simulink model "im_inv_model"  (R2026a)
settings: Solver=ode23tb  StopTime=param.sim.simlength  FixedStep=param.sim.tc  MaxStep=param.glb_time.tc  EnableMultiTasking=on
values from neighbouring files (symbols this model uses):
  param = struct()    [init_model.m]
undefined symbols (not defined in the file or in its folder): magnitude
libraries: fl_lib x53, nesl_utility x25, simulink x2, lithium_ion_battery x1, induction_machine x1, threephase_inductor_lib x1, dclink_with_center_tap x1, cstblocks_lti x1
(part 2 of 3)

== system im_inv_model/inverter//ctrl/im_ctrl/abc2dq  ==
  a : Inport
  b : Inport  Port=2
  c : Inport  Port=3
  wt : Inport  Port=4
  abc2alphabeta : Subsystem
  alphabeta2dq : Subsystem
  d : Outport  VectorParamsAs1DForOutWhenUnconnected=off
  q : Outport  Port=2  VectorParamsAs1DForOutWhenUnconnected=off
  wires:
  alphabeta2dq/2(q) -> q/1
  alphabeta2dq/1(d) -> d/1
  a/1 -> abc2alphabeta/1(a)
  c/1 -> abc2alphabeta/3(c)
  b/1 -> abc2alphabeta/2(b)
  wt/1 -> alphabeta2dq/3(wt)
  abc2alphabeta/2("beta ") -> alphabeta2dq/2(beta)
  abc2alphabeta/1("alpha ") -> alphabeta2dq/1(alpha)

== system im_inv_model/inverter//ctrl/im_ctrl/acquisition ==
  Demux1 : Demux  Outputs=3
  Gain4 : Gain  Gain=1/param.im.machine.ibez
  Gain5 : Gain  Gain=1/param.im.machine.ibez
  Gain6 : Gain  Gain=1/param.im.machine.ibez
  Quantizer1 : Quantizer  QuantizationInterval=param.meas.adc12_quantization
  Quantizer2 : Quantizer  QuantizationInterval=param.meas.adc12_quantization
  Quantizer3 : Quantizer  QuantizationInterval=param.meas.adc12_quantization
  Zero-Order Hold : ZeroOrderHold  SampleTime=param.glb_time.ts_inv
  Zero-Order Hold1 : ZeroOrderHold  SampleTime=param.glb_time.ts_inv
  Zero-Order Hold2 : ZeroOrderHold  SampleTime=param.glb_time.ts_inv
  iu : Outport  VectorParamsAs1DForOutWhenUnconnected=off
  iv : Outport  Port=2  VectorParamsAs1DForOutWhenUnconnected=off
  iw : Outport  Port=3  VectorParamsAs1DForOutWhenUnconnected=off
  wires:
  Demux1/1 -> Gain4/1
  Demux1/2 -> Gain5/1
  Demux1/3 -> Gain6/1
  [is_uvw_mod1] -> Demux1/1
  Quantizer3/1 -> Zero-Order Hold/1
  Quantizer1/1 -> Zero-Order Hold1/1
  Quantizer2/1 -> Zero-Order Hold2/1
  Gain4/1 -> Quantizer3/1
  Gain5/1 -> Quantizer1/1
  Gain6/1 -> Quantizer2/1
  Zero-Order Hold/1 -> iu/1
  Zero-Order Hold1/1 -> iv/1
  Zero-Order Hold2/1 -> iw/1

== system im_inv_model/inverter//ctrl/im_ctrl/dq2alphabeta ==
  x : Inport
  y : Inport  Port=2
  theta_s : Inport  Port=3
  dq-alphabeta : Subsystem
  dq-alphabeta1 : Subsystem
  uctrl_alpha : Outport  VectorParamsAs1DForOutWhenUnconnected=off
  uctrl_beta : Outport  Port=2  VectorParamsAs1DForOutWhenUnconnected=off
  tag scope: uctrl_alpha_mod1=global, uctrl_beta_mod1=global, ud_inv_mod1=global, uq_inv_mod1=global
  wires:
  x/1 -> dq-alphabeta/2(d), dq-alphabeta1/2(d)
  y/1 -> dq-alphabeta/3(q), dq-alphabeta1/3(q)
  theta_s/1 -> dq-alphabeta/1(wt)
  dq-alphabeta/1(alpha) -> [uctrl_alpha_mod1], uctrl_alpha/1
  dq-alphabeta/2(beta) -> [uctrl_beta_mod1], uctrl_beta/1
  [theta_slip_mod1] -> dq-alphabeta1/1(wt)
  dq-alphabeta1/1(alpha) -> [ud_inv_mod1]
  dq-alphabeta1/2(beta) -> [uq_inv_mod1]

== system im_inv_model/inverter//ctrl/im_ctrl/im_control ==
  Constant : Constant  Value=param.im.machine.alpha_norm
  Speed control : Subsystem
  Variant Source : VariantSource  VariantControls={param.im.mode.use_vector_control == 1, param.im.mode.use_uf_control == 1}
      settings: AllowZeroVariantControls=on
  Variant Source1 : VariantSource  VariantControls={param.im.mode.use_vector_control == 1, param.im.mode.use_uf_control == 1}
      settings: AllowZeroVariantControls=on
  Variant Source2 : VariantSource  VariantControls={param.im.mode.use_vector_control == 1, param.im.mode.use_uf_control == 1}
      settings: AllowZeroVariantControls=on
  current control : Subsystem
  data_analysis : Subsystem
  flux_estimator : Subsystem
  magnetization current reference : Subsystem
  speed reference : Subsystem
  u/f control : Subsystem
  usx : Outport  VectorParamsAs1DForOutWhenUnconnected=off
  usy : Outport  Port=2  VectorParamsAs1DForOutWhenUnconnected=off
  theta_s : Outport  Port=3  VectorParamsAs1DForOutWhenUnconnected=off
  tag scope: theta_s_mod1=global, torque_ref_pu_mod1=global
  wires:
  magnetization current reference/1(Ix_ref) -> current control/1(isx_ref)
  magnetization current reference/2(Iy_ref) -> current control/2(isy_ref)
  Speed control/1(torque ref) -> [torque_ref_pu_mod1]
  [omega_m_pu_mod1] -> Speed control/1(Rotor speed)
  speed reference/1(omega_m_pu_ref) -> Speed control/2(Speed ref)
  Constant/1 -> flux_estimator/1(alpha_est)
  current control/1(usx_ctrl) -> Variant Source/1
  current control/2(usy_ctrl) -> Variant Source1/1
  Variant Source/1 -> usx/1
  Variant Source1/1 -> usy/1
  u/f control/1(usx_ctrl) -> Variant Source/2
  u/f control/2(usy_ctrl) -> Variant Source1/2
  flux_estimator/1(theta_s) -> [theta_s_mod1]
  [theta_s_mod1] -> Variant Source2/1
  u/f control/3(uf_electrical_phase) -> Variant Source2/2
  Variant Source2/1 -> theta_s/1

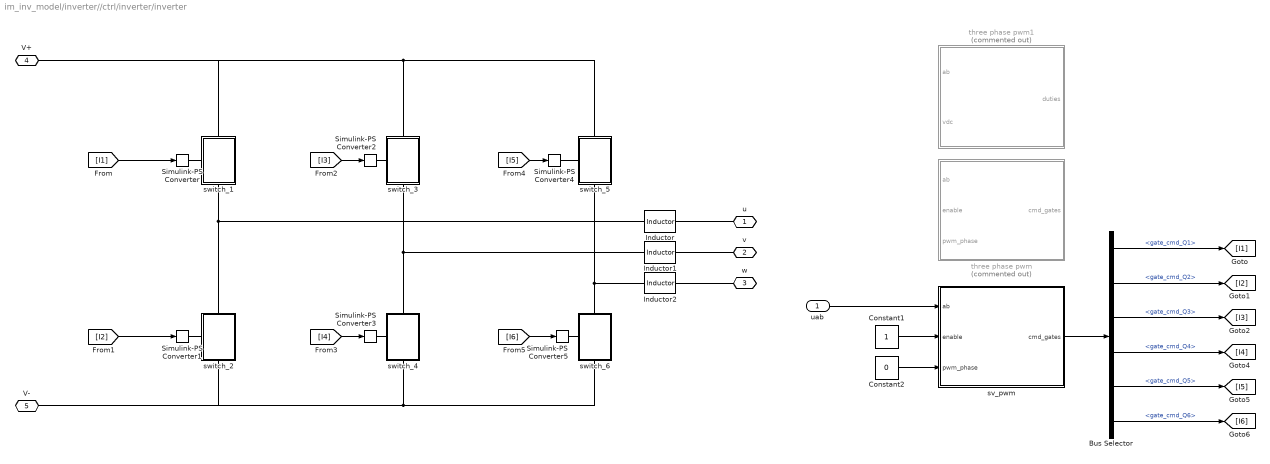
== system im_inv_model/inverter//ctrl/inverter/inverter ==
  uab : Inport
  Bus Selector : BusSelector  OutputSignals=gate_cmd_Q1,gate_cmd_Q2,gate_cmd_Q3,gate_cmd_Q4,gate_cmd_Q5,gate_cmd_Q6
  Constant1 : Constant
  Constant2 : Constant  Value=0
  Inductor : fl_lib/Electrical/Electrical Elements/Inductor  l=1e-6 H  r=0 Ohm  g=1e-9 1/Ohm  i_specify=off  i_priority=None  i=0 A  i_nominal_specify=off  i_nominal_value=1  i_nominal_unit=A  v_specify=off  v_priority=None  v=0 V  v_nominal_specify=off  v_nominal_value=1  v_nominal_unit=V  i_L_specify=off  i_L_priority=High  i_L=0 A  i_L_nominal_specify=off  i_L_nominal_value=1  i_L_nominal_unit=A
  Inductor1 : fl_lib/Electrical/Electrical Elements/Inductor  l=1e-6 H  r=0 Ohm  g=1e-9 1/Ohm  i_specify=off  i_priority=None  i=0 A  i_nominal_specify=off  i_nominal_value=1  i_nominal_unit=A  v_specify=off  v_priority=None  v=0 V  v_nominal_specify=off  v_nominal_value=1  v_nominal_unit=V  i_L_specify=off  i_L_priority=High  i_L=0 A  i_L_nominal_specify=off  i_L_nominal_value=1  i_L_nominal_unit=A
  Inductor2 : fl_lib/Electrical/Electrical Elements/Inductor  l=1e-6 H  r=0 Ohm  g=1e-9 1/Ohm  i_specify=off  i_priority=None  i=0 A  i_nominal_specify=off  i_nominal_value=1  i_nominal_unit=A  v_specify=off  v_priority=None  v=0 V  v_nominal_specify=off  v_nominal_value=1  v_nominal_unit=V  i_L_specify=off  i_L_priority=High  i_L=0 A  i_L_nominal_specify=off  i_L_nominal_value=1  i_L_nominal_unit=A
  Simulink-PS Converter{,1..5} (6 alike) : nesl_utility/Simulink-PS Converter  PhysicalDomain=network_engine_domain  SubClassName=ps_input  LeftPortType=input  RightPortType=output  PseudoPeriodic=off  Frequencies=[]  NoiseDistribution=none  NoiseParameters=[]  Unit=1  AffineConversion=on  FilteringAndDerivatives=provide  SimscapeFilterOrder=1  InputFilterTimeConstant=0.001  UdotUserProvided=0
  sv_pwm : Subsystem
  switch_1 : Subsystem
      settings: PortSchema="{\"entries\":[{\"content\":{\"sides\":[{\"content\":{\"connectorIds\":[\"LConn1\"]},\"type\":\"ConnectorPlacement.EquallySpacedRectSide\",\"uuid\":\"9277da8d-d460-43e6-8478-dd662f15d226\"},{\"content\":{\"connectorIds\":[],\"side\":\"RIGHT\"},\"type\":\"ConnectorPlacement.EquallySpacedRectSide\",\"uuid\":\"a7ece396-f1d9-4f4f-a05b-db1fc65d6e1d\"},{\"content\":{\"connectorIds\":[\"LConn2\"],\"side\":\"TOP\"},\"type\":\"ConnectorPlacement.EquallySpacedRectSide\",\"uuid\":\"fdd70777-e9cf-4317-afb6-cae87f75d5b0\"},{\"content\":{\"connectorIds\":[\"RConn1\"],\"side\":\"BOTTOM\"},\"type\":\"ConnectorPlacement.EquallySpacedRectSide\",\"uuid\":\"2353ed68-b1a1-4775-9ca9-31e268d5443b\"}]},\"type\":\"ConnectorPlacement.EquallySpacedConnector\",\"uuid\":\"d5479f4c-4e65-4791-adcb-73df11f88590\"}],\"packageUris\":[\"http://schema.mathworks.com/mf0/Connector/R2020b\"],\"version\":\"1.0\"}"
  switch_2 : Subsystem
      settings: PortSchema="{\"entries\":[{\"content\":{\"sides\":[{\"content\":{\"connectorIds\":[\"LConn1\"]},\"type\":\"ConnectorPlacement.EquallySpacedRectSide\",\"uuid\":\"9277da8d-d460-43e6-8478-dd662f15d226\"},{\"content\":{\"connectorIds\":[],\"side\":\"RIGHT\"},\"type\":\"ConnectorPlacement.EquallySpacedRectSide\",\"uuid\":\"a7ece396-f1d9-4f4f-a05b-db1fc65d6e1d\"},{\"content\":{\"connectorIds\":[\"LConn2\"],\"side\":\"TOP\"},\"type\":\"ConnectorPlacement.EquallySpacedRectSide\",\"uuid\":\"fdd70777-e9cf-4317-afb6-cae87f75d5b0\"},{\"content\":{\"connectorIds\":[\"RConn1\"],\"side\":\"BOTTOM\"},\"type\":\"ConnectorPlacement.EquallySpacedRectSide\",\"uuid\":\"2353ed68-b1a1-4775-9ca9-31e268d5443b\"}]},\"type\":\"ConnectorPlacement.EquallySpacedConnector\",\"uuid\":\"d5479f4c-4e65-4791-adcb-73df11f88590\"}],\"packageUris\":[\"http://schema.mathworks.com/mf0/Connector/R2020b\"],\"version\":\"1.0\"}"
  switch_3 : Subsystem
      settings: PortSchema="{\"entries\":[{\"content\":{\"sides\":[{\"content\":{\"connectorIds\":[\"LConn1\"]},\"type\":\"ConnectorPlacement.EquallySpacedRectSide\",\"uuid\":\"9277da8d-d460-43e6-8478-dd662f15d226\"},{\"content\":{\"connectorIds\":[],\"side\":\"RIGHT\"},\"type\":\"ConnectorPlacement.EquallySpacedRectSide\",\"uuid\":\"a7ece396-f1d9-4f4f-a05b-db1fc65d6e1d\"},{\"content\":{\"connectorIds\":[\"LConn2\"],\"side\":\"TOP\"},\"type\":\"ConnectorPlacement.EquallySpacedRectSide\",\"uuid\":\"fdd70777-e9cf-4317-afb6-cae87f75d5b0\"},{\"content\":{\"connectorIds\":[\"RConn1\"],\"side\":\"BOTTOM\"},\"type\":\"ConnectorPlacement.EquallySpacedRectSide\",\"uuid\":\"2353ed68-b1a1-4775-9ca9-31e268d5443b\"}]},\"type\":\"ConnectorPlacement.EquallySpacedConnector\",\"uuid\":\"d5479f4c-4e65-4791-adcb-73df11f88590\"}],\"packageUris\":[\"http://schema.mathworks.com/mf0/Connector/R2020b\"],\"version\":\"1.0\"}"
  switch_4 : Subsystem
      settings: PortSchema="{\"entries\":[{\"content\":{\"sides\":[{\"content\":{\"connectorIds\":[\"LConn1\"]},\"type\":\"ConnectorPlacement.EquallySpacedRectSide\",\"uuid\":\"9277da8d-d460-43e6-8478-dd662f15d226\"},{\"content\":{\"connectorIds\":[],\"side\":\"RIGHT\"},\"type\":\"ConnectorPlacement.EquallySpacedRectSide\",\"uuid\":\"a7ece396-f1d9-4f4f-a05b-db1fc65d6e1d\"},{\"content\":{\"connectorIds\":[\"LConn2\"],\"side\":\"TOP\"},\"type\":\"ConnectorPlacement.EquallySpacedRectSide\",\"uuid\":\"fdd70777-e9cf-4317-afb6-cae87f75d5b0\"},{\"content\":{\"connectorIds\":[\"RConn1\"],\"side\":\"BOTTOM\"},\"type\":\"ConnectorPlacement.EquallySpacedRectSide\",\"uuid\":\"2353ed68-b1a1-4775-9ca9-31e268d5443b\"}]},\"type\":\"ConnectorPlacement.EquallySpacedConnector\",\"uuid\":\"d5479f4c-4e65-4791-adcb-73df11f88590\"}],\"packageUris\":[\"http://schema.mathworks.com/mf0/Connector/R2020b\"],\"version\":\"1.0\"}"
  switch_5 : Subsystem
      settings: PortSchema="{\"entries\":[{\"content\":{\"sides\":[{\"content\":{\"connectorIds\":[\"LConn1\"]},\"type\":\"ConnectorPlacement.EquallySpacedRectSide\",\"uuid\":\"9277da8d-d460-43e6-8478-dd662f15d226\"},{\"content\":{\"connectorIds\":[],\"side\":\"RIGHT\"},\"type\":\"ConnectorPlacement.EquallySpacedRectSide\",\"uuid\":\"a7ece396-f1d9-4f4f-a05b-db1fc65d6e1d\"},{\"content\":{\"connectorIds\":[\"LConn2\"],\"side\":\"TOP\"},\"type\":\"ConnectorPlacement.EquallySpacedRectSide\",\"uuid\":\"fdd70777-e9cf-4317-afb6-cae87f75d5b0\"},{\"content\":{\"connectorIds\":[\"RConn1\"],\"side\":\"BOTTOM\"},\"type\":\"ConnectorPlacement.EquallySpacedRectSide\",\"uuid\":\"2353ed68-b1a1-4775-9ca9-31e268d5443b\"}]},\"type\":\"ConnectorPlacement.EquallySpacedConnector\",\"uuid\":\"d5479f4c-4e65-4791-adcb-73df11f88590\"}],\"packageUris\":[\"http://schema.mathworks.com/mf0/Connector/R2020b\"],\"version\":\"1.0\"}"
  switch_6 : Subsystem
      settings: PortSchema="{\"entries\":[{\"content\":{\"sides\":[{\"content\":{\"connectorIds\":[\"LConn1\"]},\"type\":\"ConnectorPlacement.EquallySpacedRectSide\",\"uuid\":\"9277da8d-d460-43e6-8478-dd662f15d226\"},{\"content\":{\"connectorIds\":[],\"side\":\"RIGHT\"},\"type\":\"ConnectorPlacement.EquallySpacedRectSide\",\"uuid\":\"a7ece396-f1d9-4f4f-a05b-db1fc65d6e1d\"},{\"content\":{\"connectorIds\":[\"LConn2\"],\"side\":\"TOP\"},\"type\":\"ConnectorPlacement.EquallySpacedRectSide\",\"uuid\":\"fdd70777-e9cf-4317-afb6-cae87f75d5b0\"},{\"content\":{\"connectorIds\":[\"RConn1\"],\"side\":\"BOTTOM\"},\"type\":\"ConnectorPlacement.EquallySpacedRectSide\",\"uuid\":\"2353ed68-b1a1-4775-9ca9-31e268d5443b\"}]},\"type\":\"ConnectorPlacement.EquallySpacedConnector\",\"uuid\":\"d5479f4c-4e65-4791-adcb-73df11f88590\"}],\"packageUris\":[\"http://schema.mathworks.com/mf0/Connector/R2020b\"],\"version\":\"1.0\"}"
  three phase pwm : Subsystem  Commented=on
  three phase pwm1 : Subsystem  Commented=on
  u : PMIOPort  Side=Left
  v : PMIOPort  Port=2  Side=Left
  w : PMIOPort  Port=3  Side=Left
  V+ : PMIOPort  Port=4  Side=Right
  V- : PMIOPort  Port=5  Side=Right
  wires:
  Bus Selector/6 -> [I6]  "<gate_cmd_Q6>"
  Bus Selector/5 -> [I5]  "<gate_cmd_Q5>"
  Bus Selector/4 -> [I4]  "<gate_cmd_Q4>"
  Bus Selector/3 -> [I3]  "<gate_cmd_Q3>"
  Bus Selector/2 -> [I2]  "<gate_cmd_Q2>"
  Bus Selector/1 -> [I1]  "<gate_cmd_Q1>"
  sv_pwm/1(cmd_gates) -> Bus Selector/1
  [I6] -> Simulink-PS Converter5/1
  [I5] -> Simulink-PS Converter4/1
  [I4] -> Simulink-PS Converter3/1
  [I3] -> Simulink-PS Converter2/1
  uab/1 -> sv_pwm/1(ab)
  Constant2/1 -> sv_pwm/3(pwm_phase)
  Constant1/1 -> sv_pwm/2(enable)
  [I1] -> Simulink-PS Converter/1
  [I2] -> Simulink-PS Converter1/1
  connections:
  V+/RConn1 -- switch_1/LConn2 -- switch_5/LConn2 -- switch_3/LConn2
  Inductor2/LConn1 -- switch_6/LConn2 -- switch_5/RConn1
  Inductor1/LConn1 -- switch_4/LConn2 -- switch_3/RConn1
  u/RConn1 -- Inductor/RConn1
  switch_6/LConn1 -- Simulink-PS Converter5/RConn1
  switch_5/LConn1 -- Simulink-PS Converter4/RConn1
  switch_4/LConn1 -- Simulink-PS Converter3/RConn1
  switch_3/LConn1 -- Simulink-PS Converter2/RConn1
  switch_2/LConn1 -- Simulink-PS Converter1/RConn1
  Simulink-PS Converter/RConn1 -- switch_1/LConn1
  switch_2/RConn1 -- V-/RConn1 -- switch_6/RConn1 -- switch_4/RConn1
  Inductor/LConn1 -- switch_2/LConn2 -- switch_1/RConn1
  v/RConn1 -- Inductor1/RConn1
  w/RConn1 -- Inductor2/RConn1

== system im_inv_model/inverter//ctrl/im_ctrl/abc2dq/abc2alphabeta ==
  a : Inport
  b : Inport  Port=2
  c : Inport  Port=3
  Gain1 : Gain  Gain=-1/2
  Gain11 : Gain  Gain=-1/2
  Gain2 : Gain  Gain=0
  Gain3 : Gain  Gain=sqrt(3)/2
  Gain4 : Gain  Gain=-sqrt(3)/2
  Gain8 : Gain  Gain=2/3
  Gain9 : Gain  Gain=2/3
  Sum : Sum  Inputs=+++
  Sum1 : Sum  Inputs=+++
  "alpha " : Outport  VectorParamsAs1DForOutWhenUnconnected=off
  "beta " : Outport  Port=2  VectorParamsAs1DForOutWhenUnconnected=off
  wires:
  Sum1/1 -> Gain9/1
  Sum/1 -> Gain8/1
  b/1 -> Gain11/1, Gain3/1
  c/1 -> Gain1/1, Gain4/1
  a/1 -> Sum/1, Gain2/1
  Gain4/1 -> Sum1/3
  Gain3/1 -> Sum1/2
  Gain2/1 -> Sum1/1
  Gain8/1 -> "alpha "/1
  Gain9/1 -> "beta "/1
  Gain1/1 -> Sum/3
  Gain11/1 -> Sum/2

== system im_inv_model/inverter//ctrl/im_ctrl/abc2dq/alphabeta2dq ==
  alpha : Inport
  beta : Inport  Port=2
  wt : Inport  Port=3
  Gain : Gain
  Gain1 : Gain
  Product{,1..3} (4 alike) : Product  RndMeth=Zero
  Sum : Sum
  Sum1 : Sum  Inputs=-+
  Trigonometric Function : Trigonometry  Operator=cos
  Trigonometric Function1 : Trigonometry
  d : Outport  VectorParamsAs1DForOutWhenUnconnected=off
  q : Outport  Port=2  VectorParamsAs1DForOutWhenUnconnected=off
  wires:
  [cos] -> Product/1
  alpha/1 -> Product/2, Product2/2
  Product/1 -> Sum/1
  Product1/1 -> Sum/2
  [sin] -> Product1/1
  beta/1 -> Product1/2, Product3/2
  Sum/1 -> Gain/1
  [sin] -> Product2/1
  Product2/1 -> Sum1/1
  Product3/1 -> Sum1/2
  [cos] -> Product3/1
  Sum1/1 -> Gain1/1
  Gain/1 -> d/1
  Gain1/1 -> q/1
  Trigonometric Function1/1 -> [sin]
  Trigonometric Function/1 -> [cos]
  wt/1 -> Trigonometric Function/1, Trigonometric Function1/1

== system im_inv_model/inverter//ctrl/im_ctrl/abc2dq /abc2alphabeta ==
  a : Inport
  b : Inport  Port=2
  c : Inport  Port=3
  Gain1 : Gain  Gain=-1/2
  Gain11 : Gain  Gain=-1/2
  Gain2 : Gain  Gain=0
  Gain3 : Gain  Gain=sqrt(3)/2
  Gain4 : Gain  Gain=-sqrt(3)/2
  Gain8 : Gain  Gain=2/3
  Gain9 : Gain  Gain=2/3
  Sum : Sum  Inputs=+++
  Sum1 : Sum  Inputs=+++
  "alpha " : Outport  VectorParamsAs1DForOutWhenUnconnected=off
  "beta " : Outport  Port=2  VectorParamsAs1DForOutWhenUnconnected=off
  wires:
  Gain11/1 -> Sum/2
  Gain1/1 -> Sum/3
  Gain9/1 -> "beta "/1
  Gain8/1 -> "alpha "/1
  Gain2/1 -> Sum1/1
  Gain3/1 -> Sum1/2
  Gain4/1 -> Sum1/3
  a/1 -> Gain2/1, Sum/1
  c/1 -> Gain4/1, Gain1/1
  b/1 -> Gain3/1, Gain11/1
  Sum/1 -> Gain8/1
  Sum1/1 -> Gain9/1

== system im_inv_model/inverter//ctrl/im_ctrl/abc2dq /alphabeta2dq ==
  alpha : Inport
  beta : Inport  Port=2
  wt : Inport  Port=3
  Gain : Gain
  Gain1 : Gain
  Product{,1..3} (4 alike) : Product  RndMeth=Zero
  Sum : Sum
  Sum1 : Sum  Inputs=-+
  Trigonometric Function : Trigonometry  Operator=cos
  Trigonometric Function1 : Trigonometry
  d : Outport  VectorParamsAs1DForOutWhenUnconnected=off
  q : Outport  Port=2  VectorParamsAs1DForOutWhenUnconnected=off
  wires:
  wt/1 -> Trigonometric Function1/1, Trigonometric Function/1
  Trigonometric Function/1 -> [cos]
  Trigonometric Function1/1 -> [sin]
  Gain1/1 -> q/1
  Gain/1 -> d/1
  Sum1/1 -> Gain1/1
  [cos] -> Product3/1
  Product3/1 -> Sum1/2
  Product2/1 -> Sum1/1
  [sin] -> Product2/1
  Sum/1 -> Gain/1
  beta/1 -> Product3/2, Product1/2
  [sin] -> Product1/1
  Product1/1 -> Sum/2
  Product/1 -> Sum/1
  alpha/1 -> Product2/2, Product/2
  [cos] -> Product/1

== system im_inv_model/inverter//ctrl/im_ctrl/dq2alphabeta/dq-alphabeta ==
  wt : Inport
  d : Inport  Port=2
  q : Inport  Port=3
  Product{,1..3} (4 alike) : Product  RndMeth=Zero
  Sum : Sum  Inputs=+-
  Sum1 : Sum
  Trigonometric Function : Trigonometry  Operator=cos
  Trigonometric Function1 : Trigonometry
  alpha : Outport  VectorParamsAs1DForOutWhenUnconnected=off
  beta : Outport  Port=2  VectorParamsAs1DForOutWhenUnconnected=off
  wires:
  Sum1/1 -> beta/1
  [cos] -> Product3/1
  Product3/1 -> Sum1/2
  Product2/1 -> Sum1/1
  [sin] -> Product2/1
  Sum/1 -> alpha/1
  q/1 -> Product1/2, Product3/2
  [sin] -> Product1/1
  Product1/1 -> Sum/2
  Product/1 -> Sum/1
  d/1 -> Product/2, Product2/2
  [cos] -> Product/1
  Trigonometric Function1/1 -> [sin]
  Trigonometric Function/1 -> [cos]
  wt/1 -> Trigonometric Function/1, Trigonometric Function1/1

== system im_inv_model/inverter//ctrl/im_ctrl/dq2alphabeta/dq-alphabeta1 ==
  wt : Inport
  d : Inport  Port=2
  q : Inport  Port=3
  Product{,1..3} (4 alike) : Product  RndMeth=Zero
  Sum : Sum  Inputs=+-
  Sum1 : Sum
  Trigonometric Function : Trigonometry  Operator=cos
  Trigonometric Function1 : Trigonometry
  alpha : Outport  VectorParamsAs1DForOutWhenUnconnected=off
  beta : Outport  Port=2  VectorParamsAs1DForOutWhenUnconnected=off
  wires:
  wt/1 -> Trigonometric Function1/1, Trigonometric Function/1
  Trigonometric Function/1 -> [cos]
  Trigonometric Function1/1 -> [sin]
  [cos] -> Product/1
  d/1 -> Product/2, Product2/2
  Product/1 -> Sum/1
  Product1/1 -> Sum/2
  [sin] -> Product1/1
  q/1 -> Product1/2, Product3/2
  Sum/1 -> alpha/1
  [sin] -> Product2/1
  Product2/1 -> Sum1/1
  Product3/1 -> Sum1/2
  [cos] -> Product3/1
  Sum1/1 -> beta/1

== system im_inv_model/inverter//ctrl/im_ctrl/im_control/Speed control ==
  Rotor speed : Inport
  Speed ref : Inport  Port=2
  1/Ti : Gain  Gain=param.im.ctrl.kp_w  SaturateOnIntegerOverflow=on  OutDataTypeStr=Inherit: Same as input  ParamDataTypeStr=Inherit: Same as input
  Saturation : Saturate  UpperLimit=param.im.ctrl.iq_lim  LowerLimit=-param.im.ctrl.iq_lim
  Sum1 : Sum  Inputs=+++  SaturateOnIntegerOverflow=on
  Sum2 : Sum  Inputs=-+  SaturateOnIntegerOverflow=on
  Sum3 : Sum  Inputs=-+  SaturateOnIntegerOverflow=on
  Unit Delay4 : UnitDelay  SampleTime=param.glb_time.ts_inv
  kp : Gain  Gain=param.im.ctrl.ki_w*param.glb_time.ts_inv  SaturateOnIntegerOverflow=on  OutDataTypeStr=Inherit: Same as input  ParamDataTypeStr=Inherit: Same as input
  torque ref : Outport  VectorParamsAs1DForOutWhenUnconnected=off
  wires:
  1/Ti/1 -> Sum3/1, Sum1/1
  kp/1 -> Sum1/2
  Sum2/1 -> 1/Ti/1, kp/1
  Sum1/1 -> Saturation/1
  Sum3/1 -> Unit Delay4/1
  Unit Delay4/1 -> Sum1/3
  Speed ref/1 -> Sum2/2
  Rotor speed/1 -> Sum2/1
  Saturation/1 -> torque ref/1, Sum3/2

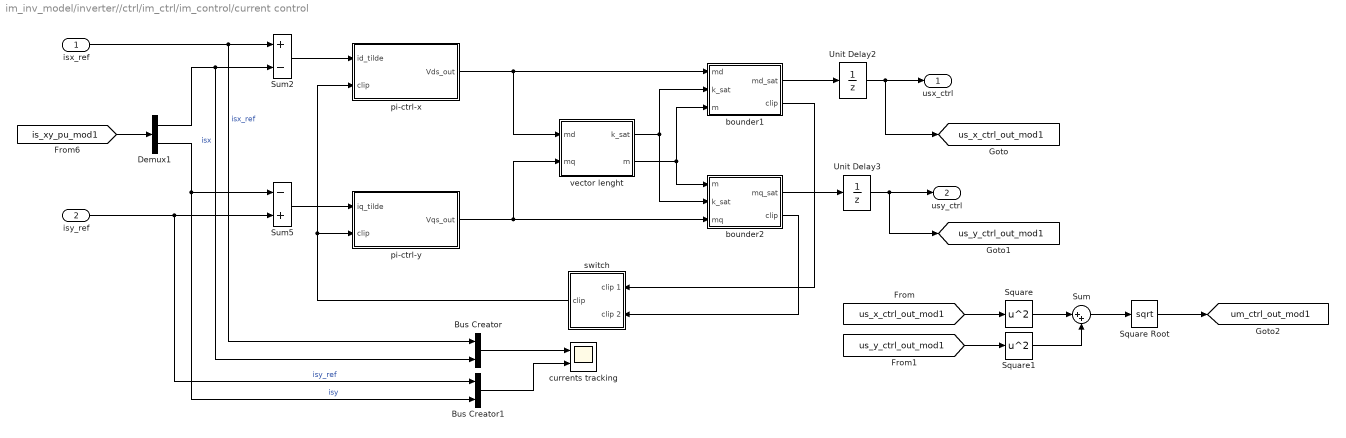
== system im_inv_model/inverter//ctrl/im_ctrl/im_control/current control ==
  isx_ref : Inport
  isy_ref : Inport  Port=2
  Bus Creator : BusCreator  Inputs=2
  Bus Creator1 : BusCreator  Inputs=2
  Demux1 : Demux  Outputs=2
  Square : Math  Operator=square
  Square Root : Sqrt
  Square1 : Math  Operator=square
  Sum : Sum  Inputs=|++
  Sum2 : Sum  Inputs=+-  SaturateOnIntegerOverflow=on
  Sum5 : Sum  Inputs=-+  SaturateOnIntegerOverflow=on
  Unit Delay2 : UnitDelay  SampleTime=param.glb_time.ts_inv
  Unit Delay3 : UnitDelay  SampleTime=param.glb_time.ts_inv
  bounder1 : Subsystem
  bounder2 : Subsystem
  currents tracking : Scope  NumInputPorts=2
      settings: ActiveDisplayYMinimum=-1  ActiveDisplayYMaximum=1
  pi-ctrl-x : Subsystem
  pi-ctrl-y : Subsystem
  switch : Subsystem
  vector lenght : Subsystem
  usx_ctrl : Outport  VectorParamsAs1DForOutWhenUnconnected=off
  usy_ctrl : Outport  Port=2  VectorParamsAs1DForOutWhenUnconnected=off
  tag scope: um_ctrl_out_mod1=global, us_x_ctrl_out_mod1=global, us_y_ctrl_out_mod1=global
  wires:
  isy_ref/1 -> Sum5/2, Bus Creator1/1  "isy_ref"
  Unit Delay3/1 -> [us_y_ctrl_out_mod1], usy_ctrl/1
  Unit Delay2/1 -> [us_x_ctrl_out_mod1], usx_ctrl/1
  [is_xy_pu_mod1] -> Demux1/1
  Demux1/2 -> Sum5/1, Bus Creator1/2  "isy"
  isx_ref/1 -> Bus Creator/1, Sum2/1  "isx_ref"
  Demux1/1 -> Bus Creator/2, Sum2/2  "isx"
  vector lenght/1(k_sat) -> bounder1/2(k_sat), bounder2/2(k_sat)
  vector lenght/2(m) -> bounder1/3(m), bounder2/1(m)
  bounder1/1(md_sat) -> Unit Delay2/1
  bounder2/1(mq_sat) -> Unit Delay3/1
  pi-ctrl-y/1(Vqs_out) -> bounder2/3(mq), vector lenght/2(mq)
  Sum5/1 -> pi-ctrl-y/1(iq_tilde)
  pi-ctrl-x/1(Vds_out) -> vector lenght/1(md), bounder1/1(md)
  switch/1(clip) -> pi-ctrl-y/2(clip), pi-ctrl-x/2(clip)
  bounder1/2(clip) -> switch/1(clip 1)
  bounder2/2(clip) -> switch/2(clip 2)
  [us_x_ctrl_out_mod1] -> Square/1
  [us_y_ctrl_out_mod1] -> Square1/1
  Square/1 -> Sum/1
  Square1/1 -> Sum/2
  Sum/1 -> Square Root/1
  Square Root/1 -> [um_ctrl_out_mod1]
  Sum2/1 -> pi-ctrl-x/1(id_tilde)
  Bus Creator/1 -> currents tracking/1
  Bus Creator1/1 -> currents tracking/2

== system im_inv_model/inverter//ctrl/im_ctrl/im_control/data_analysis ==
  double_integrator_observer_1 : Subsystem
  double_integrator_observer_2 : Subsystem
  double_integrator_observer_3 : Subsystem
  motor quantities : Scope  NumInputPorts=3
      settings: ActiveDisplayYMinimum=-0.11314190118505467  ActiveDisplayYMaximum=0.99256584414109583  DataLoggingVariableName=ScopeData2
  omega_hat : Scope  NumInputPorts=3
      settings: ActiveDisplayYMinimum=-0.50514352342653668  ActiveDisplayYMaximum=1.202582522092728
  phases_hat : Scope  NumInputPorts=3
      settings: ActiveDisplayYMinimum=-3.9269448654832364  ActiveDisplayYMaximum=3.9269536382263857  DataLoggingVariableName=ScopeData4
  speed tracking : Scope  NumInputPorts=2
      settings: ActiveDisplayYMinimum=-0.12499236282964468  ActiveDisplayYMaximum=1.1249312654668024  DataLoggingVariableName=ScopeData7
  tag scope: omega_m_mod1_hat=global, omega_s_mod1_hat=global, omega_slip_mod1_hat=global
  wires:
  [theta_m_mod1] -> phases_hat/3, double_integrator_observer_3/1(theta)  "theta_m_mod1"
  double_integrator_observer_1/1(omega_pu_hat) -> omega_hat/1, [omega_s_mod1_hat]  "omega_s_mod1_hat"
  [torque_ref_pu_mod1] -> motor quantities/3  "torque_ref"
  [is_xy_pu_mod1] -> motor quantities/1  "ixy"
  [theta_s_mod1] -> phases_hat/1, double_integrator_observer_1/1(theta)  "theta_s_mod1"
  [omega_m_pu_mod1] -> motor quantities/2  "omega_e"
  double_integrator_observer_2/1(omega_pu_hat) -> omega_hat/2, [omega_slip_mod1_hat]  "omega_slip_mod1_hat"
  double_integrator_observer_3/1(omega_pu_hat) -> omega_hat/3, [omega_m_mod1_hat]  "omega_m_mod1_hat"
  [theta_slip_mod1] -> phases_hat/2, double_integrator_observer_2/1(theta)  "theta_slip_mod1"
  [omega_m_pu_ref] -> speed tracking/2  "omega_m_pu_ref"
  [omega_m_pu_mod1] -> speed tracking/1  "omega_m_pu_mod1"

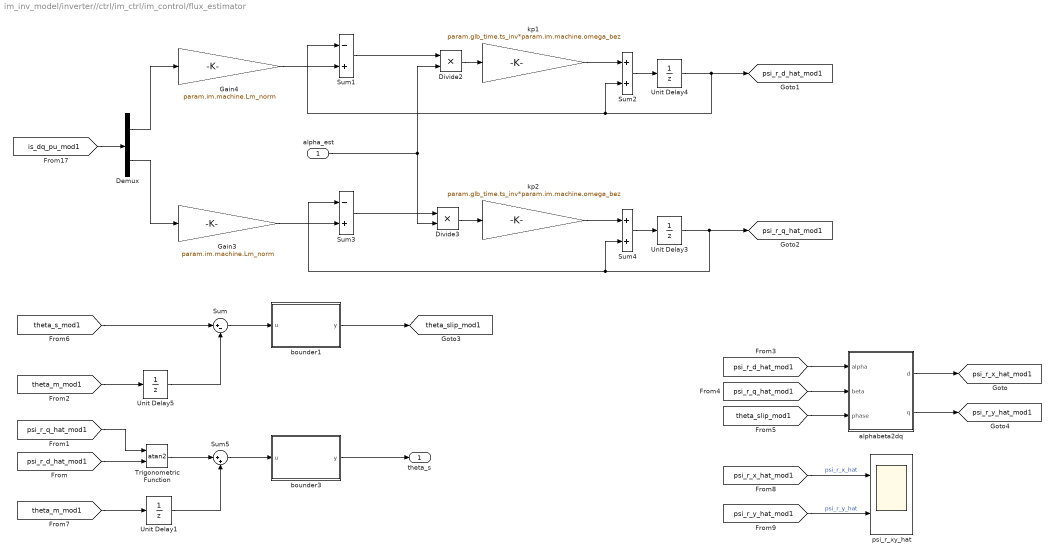
== system im_inv_model/inverter//ctrl/im_ctrl/im_control/flux_estimator ==
  alpha_est : Inport
  Demux : Demux  Outputs=2
  Divide2 : Product
  Divide3 : Product
  Gain3 : Gain  Gain=param.im.machine.Lm_norm
  Gain4 : Gain  Gain=param.im.machine.Lm_norm
  Sum : Sum  Inputs=|+-
  Sum1 : Sum  Inputs=-+  SaturateOnIntegerOverflow=on
  Sum2 : Sum  SaturateOnIntegerOverflow=on
  Sum3 : Sum  Inputs=-+  SaturateOnIntegerOverflow=on
  Sum4 : Sum  SaturateOnIntegerOverflow=on
  Sum5 : Sum  Inputs=|++
  Trigonometric Function : Trigonometry  Operator=atan2
  Unit Delay{1,3..5} (4 alike) : UnitDelay  SampleTime=param.glb_time.ts_inv
  alphabeta2dq : Subsystem
  bounder1 : MATLAB Function  TreatAsAtomicUnit=on  SystemSampleTime=param.glb_time.ts_inv
  bounder3 : MATLAB Function  TreatAsAtomicUnit=on  SystemSampleTime=param.glb_time.ts_inv
  kp1 : Gain  Gain=param.glb_time.ts_inv*param.im.machine.omega_bez  SaturateOnIntegerOverflow=on  OutDataTypeStr=Inherit: Same as input  ParamDataTypeStr=Inherit: Same as input
  kp2 : Gain  Gain=param.glb_time.ts_inv*param.im.machine.omega_bez  SaturateOnIntegerOverflow=on  OutDataTypeStr=Inherit: Same as input  ParamDataTypeStr=Inherit: Same as input
  psi_r_xy_hat : Scope  NumInputPorts=2
      settings: ActiveDisplayYMinimum=-0.32568102463349369  ActiveDisplayYMaximum=1.4062351453377793  DataLoggingVariableName=ScopeData10
  theta_s : Outport  VectorParamsAs1DForOutWhenUnconnected=off
  tag scope: psi_r_d_hat_mod1=global, psi_r_q_hat_mod1=global, psi_r_x_hat_mod1=global, psi_r_y_hat_mod1=global, theta_slip_mod1=global
  wires:
  Gain4/1 -> Sum1/2
  Unit Delay4/1 -> [psi_r_d_hat_mod1], Sum2/2, Sum1/1
  Sum1/1 -> Divide2/1
  Gain3/1 -> Sum3/2
  Unit Delay3/1 -> [psi_r_q_hat_mod1], Sum4/2, Sum3/1
  Sum3/1 -> Divide3/1
  [is_dq_pu_mod1] -> Demux/1
  Demux/1 -> Gain4/1
  Demux/2 -> Gain3/1
  [psi_r_q_hat_mod1] -> Trigonometric Function/1
  [psi_r_d_hat_mod1] -> Trigonometric Function/2
  [theta_m_mod1] -> Unit Delay5/1
  alpha_est/1 -> Divide3/2, Divide2/2
  Divide2/1 -> kp1/1
  Divide3/1 -> kp2/1
  kp1/1 -> Sum2/1
  kp2/1 -> Sum4/1
  Sum2/1 -> Unit Delay4/1
  Sum4/1 -> Unit Delay3/1
  Sum/1 -> bounder1/1(u)
  Unit Delay5/1 -> Sum/2
  [psi_r_d_hat_mod1] -> alphabeta2dq/1(alpha)
  [psi_r_q_hat_mod1] -> alphabeta2dq/2(beta)
  [theta_slip_mod1] -> alphabeta2dq/3(phase)
  alphabeta2dq/1(d) -> [psi_r_x_hat_mod1]
  alphabeta2dq/2(q) -> [psi_r_y_hat_mod1]
  [theta_s_mod1] -> Sum/1
  Trigonometric Function/1 -> Sum5/1
  [theta_m_mod1] -> Unit Delay1/1
  Unit Delay1/1 -> Sum5/2
  [psi_r_x_hat_mod1] -> psi_r_xy_hat/1  "psi_r_x_hat"
  [psi_r_y_hat_mod1] -> psi_r_xy_hat/2  "psi_r_y_hat"
  bounder1/1(y) -> [theta_slip_mod1]
  Sum5/1 -> bounder3/1(u)
  bounder3/1(y) -> theta_s/1

== system im_inv_model/inverter//ctrl/im_ctrl/im_control/magnetization current reference ==
  Bus Creator : BusCreator  Inputs=2
  Divide : Product  Inputs=*/
  Gain : Gain  Gain=1/param.im.machine.Lm_norm
  Magnitude Squared : Math  Operator=magnitude^2
  Magnitude Squared1 : Math  Operator=magnitude^2
  Magnitude Squared2 : Math  Operator=magnitude^2
  Saturation : Saturate  UpperLimit=inf  LowerLimit=1
  Sqrt : Sqrt
  Sum : Sum  Inputs=|++
  flux ctrl : Scope  NumInputPorts=2
      settings: ActiveDisplayYMinimum=-1  ActiveDisplayYMaximum=1  DataLoggingVariableName=ScopeData5
  flux ctrl1 : Scope  NumInputPorts=2
      settings: ActiveDisplayYMinimum=-1  ActiveDisplayYMaximum=1  DataLoggingVariableName=ScopeData9
  pi : Subsystem
      settings: PortSchema="{\"entries\":[{\"content\":{\"sides\":[{\"content\":{\"connectorIds\":[\"In1\",\"In2\"]},\"type\":\"ConnectorPlacement.EquallySpacedRectSide\",\"uuid\":\"c7976488-8580-40c7-ae26-3132772beaec\"},{\"content\":{\"side\":\"RIGHT\"},\"type\":\"ConnectorPlacement.EquallySpacedRectSide\",\"uuid\":\"0bf18ae2-1644-4496-bf8a-37c7109f213b\"},{\"content\":{\"side\":\"TOP\"},\"type\":\"ConnectorPlacement.EquallySpacedRectSide\",\"uuid\":\"65c43339-a6c7-4a77-b873-69b79c8b3493\"},{\"content\":{\"connectorIds\":[\"Out1\"],\"side\":\"BOTTOM\"},\"type\":\"ConnectorPlacement.EquallySpacedRectSide\",\"uuid\":\"9bf537c5-923b-4ce8-b532-4d5de915c79a\"}]},\"type\":\"ConnectorPlacement.EquallySpacedConnector\",\"uuid\":\"450bdc18-2406-48be-bad7-027766b68348\"}],\"packageUris\":[\"http://schema.mathworks.com/mf0/Connector/R2020b\"],\"version\":\"1.0\"}"
  psi_r_ref : Constant  Value=param.im.ctrl.psi_r_ref
  Ix_ref : Outport  VectorParamsAs1DForOutWhenUnconnected=off
  Iy_ref : Outport  Port=2  VectorParamsAs1DForOutWhenUnconnected=off
  tag scope: isx_ref_mod1=global, isy_ref_mod1=global
  wires:
  [torque_ref_pu_mod1] -> Iy_ref/1, [isy_ref_mod1]
  [psi_r_d_hat_mod1] -> Bus Creator/1, Magnitude Squared/1  "psi_r_d_hat_mod1"
  [psi_r_q_hat_mod1] -> Bus Creator/2, Magnitude Squared1/1  "psi_r_q_hat_mod1"
  Magnitude Squared/1 -> Sum/1
  Magnitude Squared1/1 -> Sum/2
  Sqrt/1 -> pi/1(psi_r_hat), flux ctrl1/1  "psi_r_hat"
  psi_r_ref/1 -> Divide/1
  [omega_m_pu_mod1] -> Saturation/1
  Saturation/1 -> Magnitude Squared2/1
  Divide/1 -> flux ctrl1/2, pi/2(psi_r_ref)  "psi_r_ref"
  Gain/1 -> Ix_ref/1, [isx_ref_mod1]
  Magnitude Squared2/1 -> Divide/2
  Sum/1 -> Sqrt/1
  pi/1(psi_s_ref) -> flux ctrl/2, Gain/1  "psi_s_ref"
  Bus Creator/1 -> flux ctrl/1

== system im_inv_model/inverter//ctrl/im_ctrl/im_control/speed reference ==
  1/Ti2 : Gain  Gain=1/param.im.machine.omega_m_bez  SaturateOnIntegerOverflow=on  OutDataTypeStr=Inherit: Same as input  ParamDataTypeStr=Inherit: Same as input
  LTI System : cstblocks_lti/LTI System  sys=param.im.ctrl.SOF_10Hz.ss_d  IC=[]  PadeOrder=0
  Saturation : Saturate  UpperLimit=param.im.machine.omega_m_bez  LowerLimit=0
  To Workspace7 : ToWorkspace  VariableName=omega_m_pu_ref_sim  SampleTime=param.glb_time.ts_inv
      settings: MaxDataPoints=param.glb_time.Ns_inv
  Zero-Order Hold8 : ZeroOrderHold  SampleTime=param.glb_time.ts_inv
  wref : simulink/Sources/Ramp  slope=param.im.machine.omega_m_bez  start=param.im.mode.time_start_motor_control  InitialOutput=0
  omega_m_pu_ref : Outport  VectorParamsAs1DForOutWhenUnconnected=off
  tag scope: omega_m_pu_ref=global
  wires:
  Zero-Order Hold8/1 -> 1/Ti2/1
  wref/1 -> Saturation/1
  1/Ti2/1 -> LTI System/1
  Saturation/1 -> Zero-Order Hold8/1
  LTI System/1 -> To Workspace7/1, [omega_m_pu_ref], omega_m_pu_ref/1

== system im_inv_model/inverter//ctrl/im_ctrl/im_control/u//f control ==
  Constant1 : Constant  Value=0
  Rate Limiter : RateLimiter  RisingSlewLimit=param.im.uf.uq_ref/5  FallingSlewLimit=-param.im.uf.uq_ref/5  SampleTimeMode=inherited
  Step : Step  Time=0.025  FinalValue=param.im.uf.uq_ref/5  SampleTime=0
  Step1 : Step  Time=12  FinalValue=param.im.uf.uq_ref*4/5  SampleTime=0
  Sum : Sum  Inputs=|++
  Zero-Order Hold : ZeroOrderHold  SampleTime=param.glb_time.ts_inv
  uf_phase_generation : Subsystem
  usx_ctrl : Outport  VectorParamsAs1DForOutWhenUnconnected=off
  usy_ctrl : Outport  Port=2  VectorParamsAs1DForOutWhenUnconnected=off
  uf_electrical_phase : Outport  Port=3  VectorParamsAs1DForOutWhenUnconnected=off
  wires:
  uf_phase_generation/1(uf_electrical_phase) -> uf_electrical_phase/1
  Constant1/1 -> usx_ctrl/1
  Zero-Order Hold/1 -> usy_ctrl/1
  Sum/1 -> Rate Limiter/1
  Step/1 -> Sum/1
  Step1/1 -> Sum/2
  Rate Limiter/1 -> Zero-Order Hold/1

== system im_inv_model/inverter//ctrl/inverter/inverter/sv_pwm ==
  ab : Inport
  enable : Inport  Port=2
  pwm_phase : Inport  Port=3
  -1<x<1 : Saturate  UpperLimit=1  LowerLimit=-1
  Bus Selector : BusSelector  OutputSignals=da,db,dc
  C Caller : CCaller  FunctionName=sv_pwm_process_simulink  PortSpecificationStruct="%)30     .    V @   8    (     @         %    \"     4    !     0         %  0 \"0    $    _    07)G3F%M90  4&]R=$YA;64 4V-O<&4     26YD97@     5'EP90      4VEZ90      27-';&]B86P   X    P    !@    @    $          4    (     0    ,    !         !   P!O=70 #@   #     &    \"     0         !0    @    !     P    $         $  # &]U=  .    .     8    (    !          %    \"     $    &     0         0   ...(+2669 chars)"  SampleTime=param.glb_time.ts_inv
  Constant : Constant  Value=param.glb_time.ts_inv
  Data Type Conversion1 : DataTypeConversion  OutDataTypeStr=double  SaturateOnIntegerOverflow=off  RndMeth=Floor
  Data Type Conversion15 : DataTypeConversion  OutDataTypeStr=single  SaturateOnIntegerOverflow=off  RndMeth=Floor
  Data Type Conversion16 : DataTypeConversion  OutDataTypeStr=single  SaturateOnIntegerOverflow=off  RndMeth=Floor
  Data Type Conversion17 : DataTypeConversion  OutDataTypeStr=uint32  SaturateOnIntegerOverflow=off  RndMeth=Floor
  Data Type Conversion18 : DataTypeConversion  OutDataTypeStr=single  SaturateOnIntegerOverflow=off  RndMeth=Floor
  Data Type Conversion2 : DataTypeConversion  OutDataTypeStr=double  SaturateOnIntegerOverflow=off  RndMeth=Floor
  Data Type Conversion3 : DataTypeConversion  OutDataTypeStr=double  SaturateOnIntegerOverflow=off  RndMeth=Floor
  Demux : Demux  Outputs=2
  Gain : Gain  Gain=sqrt(3)/2
  Zero-Order Hold{,1..3} (4 alike) : ZeroOrderHold  SampleTime=param.glb_time.ts_inv
  modulator1 : Subsystem
  cmd_gates : Outport
  wires:
  Demux/2 -> Data Type Conversion15/1
  ab/1 -> -1<x<1/1
  Data Type Conversion3/1 -> modulator1/3(w)  "dw"
  Bus Selector/2 -> Data Type Conversion2/1  "<db>"
  C Caller/1 -> Bus Selector/1  "out"
  Data Type Conversion17/1 -> Zero-Order Hold3/1
  Data Type Conversion15/1 -> Zero-Order Hold1/1
  Data Type Conversion2/1 -> modulator1/2(v)  "dv"
  enable/1 -> Data Type Conversion17/1
  Bus Selector/3 -> Data Type Conversion3/1  "<dc>"
  Data Type Conversion18/1 -> Zero-Order Hold/1
  Bus Selector/1 -> Data Type Conversion1/1  "<da>"
  Constant/1 -> Data Type Conversion16/1
  Data Type Conversion16/1 -> Zero-Order Hold2/1
  Zero-Order Hold/1 -> C Caller/1
  Data Type Conversion1/1 -> modulator1/1(u)  "du"
  Demux/1 -> Data Type Conversion18/1
  pwm_phase/1 -> modulator1/4(phase)
  modulator1/1(cmd_gates) -> cmd_gates/1
  Zero-Order Hold1/1 -> C Caller/2
  Zero-Order Hold2/1 -> C Caller/3
  Zero-Order Hold3/1 -> C Caller/4
  -1<x<1/1 -> Gain/1
  Gain/1 -> Demux/1

== system im_inv_model/inverter//ctrl/inverter/inverter/switch_1 ==
  Capacitor : fl_lib/Electrical/Electrical Elements/Capacitor  c=param.inv.ideal_switch.Csnubber F  r=param.inv.ideal_switch.Rsnubber Ohm  g=0 1/Ohm  i_specify=off  i_priority=None  i=0 A  i_nominal_specify=off  i_nominal_value=1  i_nominal_unit=A  v_specify=off  v_priority=None  v=0 V  v_nominal_specify=off  v_nominal_value=1  v_nominal_unit=V  vc_specify=off  vc_priority=High  vc=0 V  vc_nominal_specify=off  vc_nominal_value=1  vc_nominal_unit=V
  Diode : fl_lib/Electrical/Electrical Elements/Diode  Vf=param.inv.ideal_switch.Vdon_diode V  Ron=param.inv.ideal_switch.Rdon_diode Ohm  Goff=1e-8 1/Ohm  i_specify=off  i_priority=None  i=0 A  i_nominal_specify=off  i_nominal_value=1  i_nominal_unit=A  v_specify=off  v_priority=None  v=0 V  v_nominal_specify=off  v_nominal_value=1  v_nominal_unit=V
  Switch : fl_lib/Electrical/Electrical Elements/Switch  R_closed=param.inv.ideal_switch.Rds_on Ohm  G_open=1e-8 1/Ohm  Threshold=param.inv.ideal_switch.Vth  i_specify=off  i_priority=None  i=0 A  i_nominal_specify=off  i_nominal_value=1  i_nominal_unit=A  v_specify=off  v_priority=None  v=0 V  v_nominal_specify=off  v_nominal_value=1  v_nominal_unit=V
  G : PMIOPort  Side=Left
  C : PMIOPort  Port=2  Side=Left
  E : PMIOPort  Port=3  Side=Right
  connections:
  E/RConn1 -- Switch/LConn1 -- Capacitor/RConn1 -- Diode/LConn1
  Switch/RConn1 -- G/RConn1
  C/RConn1 -- Switch/RConn2 -- Capacitor/LConn1 -- Diode/RConn1

== system im_inv_model/inverter//ctrl/inverter/inverter/switch_2 ==
  Capacitor : fl_lib/Electrical/Electrical Elements/Capacitor  c=param.inv.ideal_switch.Csnubber F  r=param.inv.ideal_switch.Rsnubber Ohm  g=0 1/Ohm  i_specify=off  i_priority=None  i=0 A  i_nominal_specify=off  i_nominal_value=1  i_nominal_unit=A  v_specify=off  v_priority=None  v=0 V  v_nominal_specify=off  v_nominal_value=1  v_nominal_unit=V  vc_specify=off  vc_priority=High  vc=0 V  vc_nominal_specify=off  vc_nominal_value=1  vc_nominal_unit=V
  Diode : fl_lib/Electrical/Electrical Elements/Diode  Vf=param.inv.ideal_switch.Vdon_diode V  Ron=param.inv.ideal_switch.Rdon_diode Ohm  Goff=1e-8 1/Ohm  i_specify=off  i_priority=None  i=0 A  i_nominal_specify=off  i_nominal_value=1  i_nominal_unit=A  v_specify=off  v_priority=None  v=0 V  v_nominal_specify=off  v_nominal_value=1  v_nominal_unit=V
  Switch : fl_lib/Electrical/Electrical Elements/Switch  R_closed=param.inv.ideal_switch.Rds_on Ohm  G_open=1e-8 1/Ohm  Threshold=param.inv.ideal_switch.Vth  i_specify=off  i_priority=None  i=0 A  i_nominal_specify=off  i_nominal_value=1  i_nominal_unit=A  v_specify=off  v_priority=None  v=0 V  v_nominal_specify=off  v_nominal_value=1  v_nominal_unit=V
  G : PMIOPort  Side=Left
  C : PMIOPort  Port=2  Side=Left
  E : PMIOPort  Port=3  Side=Right
  connections:
  Diode/RConn1 -- Capacitor/LConn1 -- Switch/RConn2 -- C/RConn1
  Switch/RConn1 -- G/RConn1
  Diode/LConn1 -- Capacitor/RConn1 -- Switch/LConn1 -- E/RConn1

== system im_inv_model/inverter//ctrl/inverter/inverter/switch_3 ==
  Capacitor : fl_lib/Electrical/Electrical Elements/Capacitor  c=param.inv.ideal_switch.Csnubber F  r=param.inv.ideal_switch.Rsnubber Ohm  g=0 1/Ohm  i_specify=off  i_priority=None  i=0 A  i_nominal_specify=off  i_nominal_value=1  i_nominal_unit=A  v_specify=off  v_priority=None  v=0 V  v_nominal_specify=off  v_nominal_value=1  v_nominal_unit=V  vc_specify=off  vc_priority=High  vc=0 V  vc_nominal_specify=off  vc_nominal_value=1  vc_nominal_unit=V
  Diode : fl_lib/Electrical/Electrical Elements/Diode  Vf=param.inv.ideal_switch.Vdon_diode V  Ron=param.inv.ideal_switch.Rdon_diode Ohm  Goff=1e-8 1/Ohm  i_specify=off  i_priority=None  i=0 A  i_nominal_specify=off  i_nominal_value=1  i_nominal_unit=A  v_specify=off  v_priority=None  v=0 V  v_nominal_specify=off  v_nominal_value=1  v_nominal_unit=V
  Switch : fl_lib/Electrical/Electrical Elements/Switch  R_closed=param.inv.ideal_switch.Rds_on Ohm  G_open=1e-8 1/Ohm  Threshold=param.inv.ideal_switch.Vth  i_specify=off  i_priority=None  i=0 A  i_nominal_specify=off  i_nominal_value=1  i_nominal_unit=A  v_specify=off  v_priority=None  v=0 V  v_nominal_specify=off  v_nominal_value=1  v_nominal_unit=V
  G : PMIOPort  Side=Left
  C : PMIOPort  Port=2  Side=Left
  E : PMIOPort  Port=3  Side=Right
  connections:
  E/RConn1 -- Switch/LConn1 -- Capacitor/RConn1 -- Diode/LConn1
  Switch/RConn1 -- G/RConn1
  C/RConn1 -- Switch/RConn2 -- Capacitor/LConn1 -- Diode/RConn1

== system im_inv_model/inverter//ctrl/inverter/inverter/switch_4 ==
  Capacitor : fl_lib/Electrical/Electrical Elements/Capacitor  c=param.inv.ideal_switch.Csnubber F  r=param.inv.ideal_switch.Rsnubber Ohm  g=0 1/Ohm  i_specify=off  i_priority=None  i=0 A  i_nominal_specify=off  i_nominal_value=1  i_nominal_unit=A  v_specify=off  v_priority=None  v=0 V  v_nominal_specify=off  v_nominal_value=1  v_nominal_unit=V  vc_specify=off  vc_priority=High  vc=0 V  vc_nominal_specify=off  vc_nominal_value=1  vc_nominal_unit=V
  Diode : fl_lib/Electrical/Electrical Elements/Diode  Vf=param.inv.ideal_switch.Vdon_diode V  Ron=param.inv.ideal_switch.Rdon_diode Ohm  Goff=1e-8 1/Ohm  i_specify=off  i_priority=None  i=0 A  i_nominal_specify=off  i_nominal_value=1  i_nominal_unit=A  v_specify=off  v_priority=None  v=0 V  v_nominal_specify=off  v_nominal_value=1  v_nominal_unit=V
  Switch : fl_lib/Electrical/Electrical Elements/Switch  R_closed=param.inv.ideal_switch.Rds_on Ohm  G_open=1e-8 1/Ohm  Threshold=param.inv.ideal_switch.Vth  i_specify=off  i_priority=None  i=0 A  i_nominal_specify=off  i_nominal_value=1  i_nominal_unit=A  v_specify=off  v_priority=None  v=0 V  v_nominal_specify=off  v_nominal_value=1  v_nominal_unit=V
  G : PMIOPort  Side=Left
  C : PMIOPort  Port=2  Side=Left
  E : PMIOPort  Port=3  Side=Right
  connections:
  Diode/RConn1 -- Capacitor/LConn1 -- Switch/RConn2 -- C/RConn1
  Switch/RConn1 -- G/RConn1
  Diode/LConn1 -- Capacitor/RConn1 -- Switch/LConn1 -- E/RConn1

== system im_inv_model/inverter//ctrl/inverter/inverter/switch_5 ==
  Capacitor : fl_lib/Electrical/Electrical Elements/Capacitor  c=param.inv.ideal_switch.Csnubber F  r=param.inv.ideal_switch.Rsnubber Ohm  g=0 1/Ohm  i_specify=off  i_priority=None  i=0 A  i_nominal_specify=off  i_nominal_value=1  i_nominal_unit=A  v_specify=off  v_priority=None  v=0 V  v_nominal_specify=off  v_nominal_value=1  v_nominal_unit=V  vc_specify=off  vc_priority=High  vc=0 V  vc_nominal_specify=off  vc_nominal_value=1  vc_nominal_unit=V
  Diode : fl_lib/Electrical/Electrical Elements/Diode  Vf=param.inv.ideal_switch.Vdon_diode V  Ron=param.inv.ideal_switch.Rdon_diode Ohm  Goff=1e-8 1/Ohm  i_specify=off  i_priority=None  i=0 A  i_nominal_specify=off  i_nominal_value=1  i_nominal_unit=A  v_specify=off  v_priority=None  v=0 V  v_nominal_specify=off  v_nominal_value=1  v_nominal_unit=V
  Switch : fl_lib/Electrical/Electrical Elements/Switch  R_closed=param.inv.ideal_switch.Rds_on Ohm  G_open=1e-8 1/Ohm  Threshold=param.inv.ideal_switch.Vth  i_specify=off  i_priority=None  i=0 A  i_nominal_specify=off  i_nominal_value=1  i_nominal_unit=A  v_specify=off  v_priority=None  v=0 V  v_nominal_specify=off  v_nominal_value=1  v_nominal_unit=V
  G : PMIOPort  Side=Left
  C : PMIOPort  Port=2  Side=Left
  E : PMIOPort  Port=3  Side=Right
  connections:
  E/RConn1 -- Switch/LConn1 -- Capacitor/RConn1 -- Diode/LConn1
  Switch/RConn1 -- G/RConn1
  C/RConn1 -- Switch/RConn2 -- Capacitor/LConn1 -- Diode/RConn1

== system im_inv_model/inverter//ctrl/inverter/inverter/switch_6 ==
  Capacitor : fl_lib/Electrical/Electrical Elements/Capacitor  c=param.inv.ideal_switch.Csnubber F  r=param.inv.ideal_switch.Rsnubber Ohm  g=0 1/Ohm  i_specify=off  i_priority=None  i=0 A  i_nominal_specify=off  i_nominal_value=1  i_nominal_unit=A  v_specify=off  v_priority=None  v=0 V  v_nominal_specify=off  v_nominal_value=1  v_nominal_unit=V  vc_specify=off  vc_priority=High  vc=0 V  vc_nominal_specify=off  vc_nominal_value=1  vc_nominal_unit=V
  Diode : fl_lib/Electrical/Electrical Elements/Diode  Vf=param.inv.ideal_switch.Vdon_diode V  Ron=param.inv.ideal_switch.Rdon_diode Ohm  Goff=1e-8 1/Ohm  i_specify=off  i_priority=None  i=0 A  i_nominal_specify=off  i_nominal_value=1  i_nominal_unit=A  v_specify=off  v_priority=None  v=0 V  v_nominal_specify=off  v_nominal_value=1  v_nominal_unit=V
  Switch : fl_lib/Electrical/Electrical Elements/Switch  R_closed=param.inv.ideal_switch.Rds_on Ohm  G_open=1e-8 1/Ohm  Threshold=param.inv.ideal_switch.Vth  i_specify=off  i_priority=None  i=0 A  i_nominal_specify=off  i_nominal_value=1  i_nominal_unit=A  v_specify=off  v_priority=None  v=0 V  v_nominal_specify=off  v_nominal_value=1  v_nominal_unit=V
  G : PMIOPort  Side=Left
  C : PMIOPort  Port=2  Side=Left
  E : PMIOPort  Port=3  Side=Right
  connections:
  Diode/RConn1 -- Capacitor/LConn1 -- Switch/RConn2 -- C/RConn1
  Switch/RConn1 -- G/RConn1
  Diode/LConn1 -- Capacitor/RConn1 -- Switch/LConn1 -- E/RConn1

== system im_inv_model/inverter//ctrl/inverter/inverter/three phase pwm ==
  ab : Inport
  enable : Inport  Port=2
  pwm_phase : Inport  Port=3
  Constant : Constant  Value=sqrt(3)/2
  Demux1 : Demux  Outputs=2
  Gain1 : Gain  Gain=1/sqrt(3)
  Gain2 : Gain  Gain=1/sqrt(3)
  Gain3 : Gain  Gain=1/sqrt(3)
  Sum : Sum  Inputs=|+-
  Sum1 : Sum  Inputs=|+-
  Sum2 : Sum  Inputs=|+-
  Sum3 : Sum  Inputs=|++
  Sum4 : Sum  Inputs=|++
  Sum5 : Sum  Inputs=|++
  Third harmonic injecting : Subsystem
  modulator : Subsystem
  uvw2alphabeta1 : MATLAB Function  TreatAsAtomicUnit=on  SystemSampleTime=param.glb_time.ts_inv
  cmd_gates : Outport
  wires:
  uvw2alphabeta1/3(w) -> Third harmonic injecting/3(m3), Sum2/1  "wr"
  uvw2alphabeta1/2(v) -> Sum1/1, Third harmonic injecting/2(m2)  "vr"
  uvw2alphabeta1/1(u) -> Sum/1, Third harmonic injecting/1(m1)  "ur"
  Third harmonic injecting/1(trn) -> Sum2/2, Sum/2, Sum1/2
  Demux1/2 -> uvw2alphabeta1/2(beta)
  Demux1/1 -> uvw2alphabeta1/1(alpha)
  ab/1 -> Demux1/1
  Sum/1 -> Sum3/1
  Sum3/1 -> Gain3/1
  Sum1/1 -> Sum4/1
  Sum2/1 -> Sum5/1
  Constant/1 -> Sum3/2, Sum4/2, Sum5/2
  Gain3/1 -> modulator/1(u)
  Sum4/1 -> Gain1/1
  Sum5/1 -> Gain2/1
  Gain1/1 -> modulator/2(v)
  Gain2/1 -> modulator/3(w)
  pwm_phase/1 -> modulator/4(phase)
  modulator/1(cmd_gates) -> cmd_gates/1

== system im_inv_model/inverter//ctrl/inverter/inverter/three phase pwm1 ==
  ab : Inport
  vdc : Inport  Port=2
  Bus Creator : BusCreator  Inputs=2
  Bus Creator1 : BusCreator  Inputs=2
  Bus Creator2 : BusCreator  Inputs=2
  Bus Creator3 : BusCreator  Inputs=3
  Demux1 : Demux  Outputs=2
  Divide : Product  Inputs=/*
  Divide1 : Product  Inputs=/*
  Divide2 : Product  Inputs=/*
  Gain6 : Gain  Gain=1/sqrt(3)*2
  Gain7 : Gain  Gain=1/sqrt(3)*2
  Gain8 : Gain  Gain=1/sqrt(3)*2
  PWM generator 1 : Subsystem  mask{f=param.glb_time.fPWM_INV, ph=0, m_up=1, m_low=-1, dead_time=0}
      mask prompts: f "Frequency"; ph "Phase"; m_up "Max Input Modulation Value"; m_low "Min Input Modulation Value"; dead_time "Dead Time"
  PWM generator 2 : Subsystem  mask{f=param.glb_time.fPWM_INV, ph=0, m_up=1, m_low=-1, dead_time=0}
      mask prompts: f "Frequency"; ph "Phase"; m_up "Max Input Modulation Value"; m_low "Min Input Modulation Value"; dead_time "Dead Time"
  PWM generator 3 : Subsystem  mask{f=param.glb_time.fPWM_INV, ph=0, m_up=1, m_low=-1, dead_time=0}
      mask prompts: f "Frequency"; ph "Phase"; m_up "Max Input Modulation Value"; m_low "Min Input Modulation Value"; dead_time "Dead Time"
  Sum : Sum  Inputs=|+-
  Sum1 : Sum  Inputs=|+-
  Sum2 : Sum  Inputs=|+-
  Third harmonic injecting : Subsystem
  uvw2alphabeta1 : MATLAB Function  TreatAsAtomicUnit=on  SystemSampleTime=param.glb_time.ts_inv
  duties : Outport
  wires:
  ab/1 -> Demux1/1
  Demux1/1 -> uvw2alphabeta1/1(alpha)
  Demux1/2 -> uvw2alphabeta1/2(beta)
  Third harmonic injecting/1(thind_H) -> Sum1/2, Sum/2, Sum2/2
  uvw2alphabeta1/1(u) -> Third harmonic injecting/1(m1), Sum/1  "ur"
  uvw2alphabeta1/2(v) -> Third harmonic injecting/2(m2), Sum1/1  "vr"
  uvw2alphabeta1/3(w) -> Sum2/1, Third harmonic injecting/3(m3)  "wr"
  vdc/1 -> Divide2/1, Divide1/1, Divide/1
  Sum/1 -> Gain6/1
  Divide/1 -> PWM generator 1/1(m_index)
  Divide2/1 -> PWM generator 3/1(m_index)
  Divide1/1 -> PWM generator 2/1(m_index)
  PWM generator 1/1(m1) -> Bus Creator/1  "gate_cmd_Q1"
  PWM generator 2/1(m1) -> Bus Creator1/1  "gate_cmd_Q3"
  PWM generator 3/1(m1) -> Bus Creator2/1  "gate_cmd_Q5"
  Bus Creator3/1 -> duties/1
  PWM generator 1/2(m2) -> Bus Creator/2  "gate_cmd_Q2"
  PWM generator 2/2(m2) -> Bus Creator1/2  "gate_cmd_Q4"
  PWM generator 3/2(m2) -> Bus Creator2/2  "gate_cmd_Q6"
  Bus Creator1/1 -> Bus Creator3/2  "gate_cmd_leg_v"
  Bus Creator/1 -> Bus Creator3/1  "gate_cmd_leg_u"
  Bus Creator2/1 -> Bus Creator3/3  "gate_cmd_leg_w"
  Gain6/1 -> Divide/2
  Sum1/1 -> Gain7/1
  Sum2/1 -> Gain8/1
  Gain7/1 -> Divide1/2
  Gain8/1 -> Divide2/2
